simulink model "OCC_DQ_RCC_PO_BOOST_COMMON_GROUND_UPM"  (R2023a)
settings: Solver=ode1  StartTime=0.0  StopTime=5  FixedStep=1e-6  MaxStep=1e-6  RelTol=1e-3  EnableMultiTasking=on
undefined symbols (not defined in the file or in its folder): DiscIntNeverNeededParam
libraries: simulink x15, spsSeriesRLCBranchLib x14, spsVoltageMeasurementLib x8, slpidlib x7, spsDiodeLib x6, spsFirstOrderFilterLib x6, spsMosfetLib x5, powerlib_extras x5, spsCurrentMeasurementLib x4, spsAlphaBetaZerotodq0Lib x3, eePowerMeasurement x2, spsACVoltageSourceLib x1
(part 1 of 2)
Description:
  | Model of a simple control system for use iin training.
settings Model: Creator=Paul Baracos  LastModifiedBy=RAGHAVA
settings SolverCC: AutoInsertRateTranBlk=on
settings DataIOCC: LimitDataPoints=on  SaveFormat=StructureWithTime  SignalLoggingSaveFormat=ModelDataLogs  SaveOutput=off  SaveTime=off  ReturnWorkspaceOutputs=off  SignalLoggingName=sigsOut
settings OptimizationCC: BlockReduction=off  BooleanDataType=off  OptimizeBlockIOStorage=off  BufferReuse=off  ExpressionFolding=off  ExpressionDepthLimit=2147483647  LocalBlockOutputs=off  InitFltsAndDblsToZero=on  LifeSpan=inf
settings DebuggingCC: SaveWithParameterizedLinksMsg=none  UnderspecifiedInitializationDetection=Classic  MergeDetectMultiDrivingBlocksExec=none  SignalResolutionControl=TryResolveAllWithWarning  MultiTaskDSMMsg=warning  MultiTaskCondExecSysMsg=none  FcnCallInpInsideContextMsg=warning  UnconnectedInputMsg=warning  UnconnectedOutputMsg=warning  UnconnectedLineMsg=warning  StateNameClashWarn=warning  SFUnexpectedBacktrackingDiag=warning  SFNoUnconditionalDefaultTransitionDiag=warning  SFExecutionAtInitializationDiag=none  ArithmeticOperatorsInVariantConditions=warning
settings HardwareCC: ProdBitPerPointer=32  ProdBitPerSizeT=32  ProdBitPerPtrDiffT=32  ProdLargestAtomicFloat=None  ProdIntDivRoundTo=Undefined  ProdEndianess=Unspecified  ProdWordSize=32  ProdHWDeviceType=32-bit Generic  TargetBitPerPointer=64  TargetBitPerSizeT=64  TargetBitPerPtrDiffT=64  TargetLongLongMode=on  TargetIntDivRoundTo=Zero  TargetEndianess=LittleEndian  TargetWordSize=64  TargetHWDeviceType=MATLAB Host  ProdEqTarget=off
settings ModelReferenceCC: PropagateSignalLabelsOutOfModel=off
settings SFSimCC: SimUseLocalCustomCode=off  CustomCodeUndefinedFunction=UseInterfaceOnly
settings RTWCC: RTWUseLocalCustomCode=off
settings CodeAppCC: StateflowObjectComments=on
settings GRTTargetCC: TargetFcnLib=ansi_tfl_tmw.mat  TargetLangStandard=C89/C90 (ANSI)  CombineOutputUpdateFcns=off  GRTInterface=on
settings ConfigComp: CovMetricSettings=dw  CovSaveCumulativeToWorkspaceVar=on  CovSaveSingleToWorkspaceVar=on  CovExternalEMLEnable=off

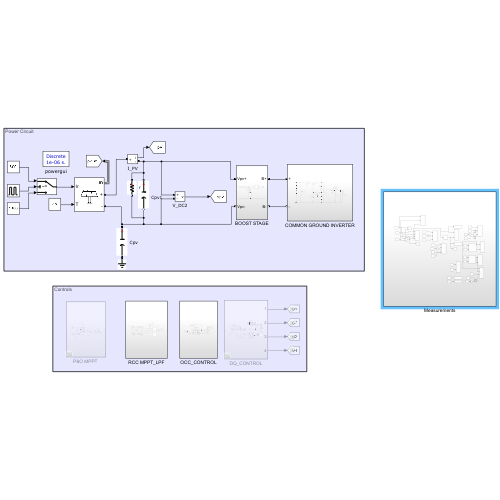
[thumbnail: Simulink's stored preview of the top-level diagram]
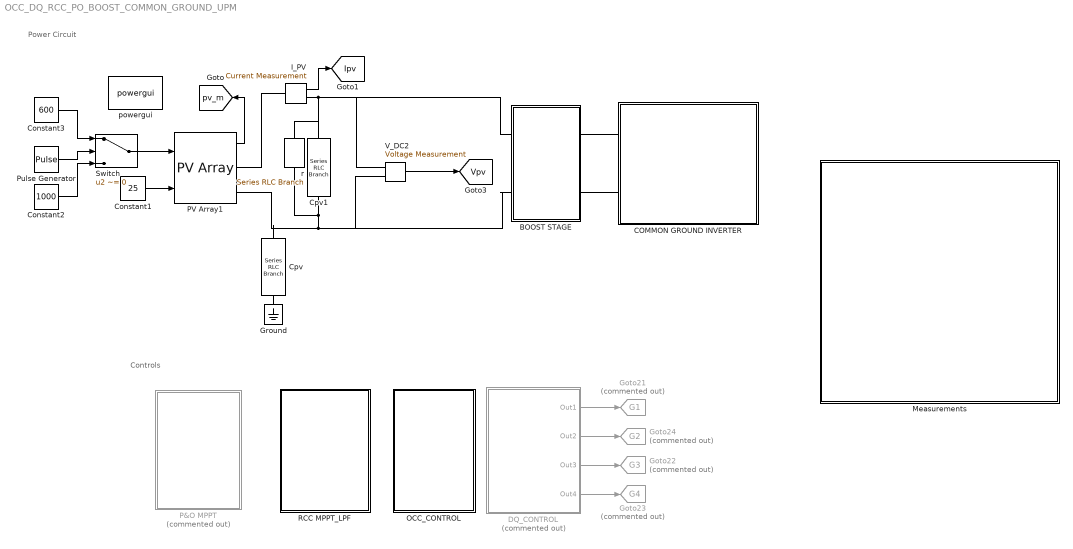
== system OCC_DQ_RCC_PO_BOOST_COMMON_GROUND_UPM ==
  note: Controls
  note: Power Circuit
  " Cpv1" : spsSeriesRLCBranchLib/Series RLC Branch  LConnTagsString=__new0  RConnTagsString=__new0  BranchType=C  Resistance=1  Inductance=15.5e-3  SetiL0=off  InitialCurrent=0  Capacitance=10e-6  Setx0=on  InitialVoltage=130  Measurements=Branch voltage and current
  BOOST STAGE : Subsystem
  COMMON GROUND INVERTER : Subsystem
  Constant1 : Constant  Value=25  SampleTime=0
  Constant2 : Constant  Value=1000
  Constant3 : Constant  Value=600
  Cpv : spsSeriesRLCBranchLib/Series RLC Branch  LConnTagsString=__new0  RConnTagsString=__new0  BranchType=C  Resistance=0.0001  Inductance=15.5e-3  SetiL0=off  InitialCurrent=0  Capacitance=100e-9  Setx0=off  InitialVoltage=0  Measurements=Branch voltage and current
  DQ_CONTROL : Subsystem  Commented=on
  Goto21 : Goto  Commented=on  GotoTag=G1  TagVisibility=global
  Goto22 : Goto  Commented=on  GotoTag=G3  TagVisibility=global
  Goto23 : Goto  Commented=on  GotoTag=G4  TagVisibility=global
  Goto24 : Goto  Commented=on  GotoTag=G2  TagVisibility=global
  Ground : spsGroundLib/Ground  LConnTagsString=a
  I_PV : spsCurrentMeasurementLib/Current Measurement  PhasorSimulation=off  OutputType=Complex  PSBequivalent=0
  Measurements : Subsystem
  OCC_CONTROL : Subsystem
  "P&O MPPT " : Subsystem  Commented=on
  PV Array1 : spsPVArrayLib/PV Array  Npar=1  Nser=5  PlotType=array @ 25 deg.C & specified irradiances  S_vec="[ 1000  600  100 ]"  Temp_C_vec="[ 45 25  ]"  ModuleName=Kyocera Solar KC200GT  PlotWhenSelected=off  Pm=200.143  Ncell=54  Voc=32.9  Isc=8.21  Vm=26.3  Im=7.61  beta_Voc_pc=-0.355  alpha_Isc_pc=0.06  beta_Voc=-0.11679  alpha_Isc=0.004926  IL=8.2288  I0=2.3234e-10  nI=0.97734  Rsh=150.6844  Rs=0.34484  RobustModel=off  RobustCellTemperature=313.3991  BAL=on  Tc=1e-6  Tfilter=5e-5
  Pulse Generator : DiscretePulseGenerator  PulseType=Time based  PulseWidth=50
  RCC MPPT_LPF : Subsystem
  Switch : Switch  Criteria=u2 ~= 0  SaturateOnIntegerOverflow=off  InputSameDT=off
  V_DC2 : spsVoltageMeasurementLib/Voltage Measurement  PhasorSimulation=off  OutputType=Complex  PSBequivalent=0
  powergui : sps_lib/powergui  Priority=1  SimulationMode=Discrete  SampleTime=1e-6  frequency=60  Iterations=50  frequencyindice=0  Pbase=100e6  ErrMax=1e-4  UnitsV=kV  UnitsW=MW  buscounter=0  FunctionMessages=off  echomessages=off  EnableUseOfTLC=off  CurrentSourceSwitches=off  DisableSnubberDevices=on  DisableRonSwitches=on  DisableVfSwitches=on  DisplayEquations=off  AutomaticDiscreteSolvers=off  SolverType=Tustin/Backward Euler (TBE)  Interpol=off  ExternalGateDelay=off  methode=off  Ts=0  x0status=blocks  SPID=on  SwTol=0  HookPort=off  NonlinearTolerance=1e-4  nMaxIteration=100  ContinueOnMaxIteration=off  RestoreLinks=warning  ResistiveCurrentMeasurement=off  Frange=[0:2:500]  Ylog=off  Xlog=on  ShowGrid=off  save=off  variable=ZData  structure=0  ZoomFFT=off  StartTime=0.0  cycles=1  DisplayStyle=1  fundamental=60  FreqAxis=off  MaxFrequency=1000  frequencyindicesteady=1  RmsSteady=1  display=off
  r : spsSeriesRLCBranchLib/Series RLC Branch  LConnTagsString=__new0  RConnTagsString=__new0  BranchType=R  Resistance=10000  Inductance=15.5e-3  SetiL0=off  InitialCurrent=0  Capacitance=2200e-6  Setx0=off  InitialVoltage=0  Measurements=Branch voltage and current
  tag scope: Ipv=global, Vpv=global, pv_m=global
  wires:
  Pulse Generator/1 -> Switch/2
  I_PV/1 -> [Ipv]
  Constant1/1 -> PV Array1/2
  V_DC2/1 -> [Vpv]
  PV Array1/1 -> [pv_m]
  DQ_CONTROL/3(Out3) -> Goto22/1
  DQ_CONTROL/2(Out2) -> Goto24/1
  DQ_CONTROL/4(Out4) -> Goto23/1
  DQ_CONTROL/1(Out1) -> Goto21/1
  Constant2/1 -> Switch/3
  Constant3/1 -> Switch/1
  Switch/1 -> PV Array1/1
  connections:
  PV Array1/RConn1 -- I_PV/LConn1
  I_PV/RConn1 -- r/LConn1 -- " Cpv1"/LConn1 -- V_DC2/LConn1 -- BOOST STAGE/LConn1
  " Cpv1"/RConn1 -- r/RConn1 -- Cpv/LConn1 -- PV Array1/RConn2 -- V_DC2/LConn2 -- BOOST STAGE/LConn2
  COMMON GROUND INVERTER/LConn1 -- BOOST STAGE/RConn1
  COMMON GROUND INVERTER/LConn2 -- BOOST STAGE/RConn2
  Ground/LConn1 -- Cpv/RConn1

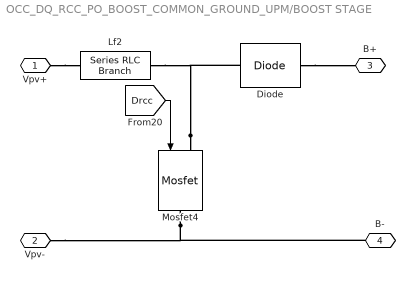
== system OCC_DQ_RCC_PO_BOOST_COMMON_GROUND_UPM/BOOST STAGE ==
  Diode : spsDiodeLib/Diode  Ron=0.001  Lon=0  Vf=0.8  IC=0  UseSnubber=0  Rs=500  Cs=250e-9  Measurements=off
  Lf2 : spsSeriesRLCBranchLib/Series RLC Branch  LConnTagsString=__new0  RConnTagsString=__new0  BranchType=RL  Resistance=0.0001  Inductance=5.87e-3  SetiL0=off  InitialCurrent=0  Capacitance=1e-6  Setx0=off  InitialVoltage=0  Measurements=Branch voltage and current
  Mosfet4 : spsMosfetLib/Mosfet  Ron=0.001  Lon=0  Rd=0.001  Vfd=0.8  IC=0  Rs=1e9  Cs=inf  Measurements=off
  Vpv+ : PMIOPort  Side=Left
  Vpv- : PMIOPort  Port=2  Side=Left
  B+ : PMIOPort  Port=3  Side=Right
  B- : PMIOPort  Port=4  Side=Right
  wires:
  [Drcc] -> Mosfet4/1
  connections:
  Diode/RConn1 -- B+/RConn1
  Vpv+/RConn1 -- Lf2/LConn1
  Mosfet4/RConn1 -- B-/RConn1 -- Vpv-/RConn1
  Mosfet4/LConn1 -- Diode/LConn1 -- Lf2/RConn1

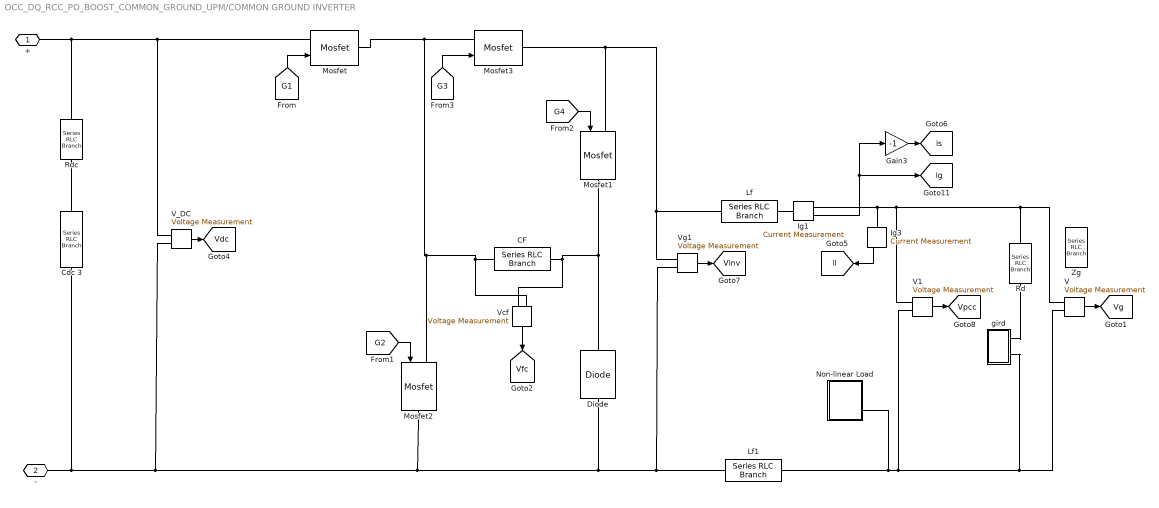
== system OCC_DQ_RCC_PO_BOOST_COMMON_GROUND_UPM/COMMON GROUND INVERTER ==
  CF : spsSeriesRLCBranchLib/Series RLC Branch  LConnTagsString=__new0  RConnTagsString=__new0  BranchType=C  Resistance=0.0001  Inductance=15.5e-3  SetiL0=off  InitialCurrent=0  Capacitance=1100e-6  Setx0=on  InitialVoltage=400  Measurements=Branch voltage and current
  Cdc 3 : spsSeriesRLCBranchLib/Series RLC Branch  LConnTagsString=__new0  RConnTagsString=__new0  BranchType=C  Resistance=0.0001  Inductance=15.5e-3  SetiL0=off  InitialCurrent=0  Capacitance=1000e-6  Setx0=on  InitialVoltage=400  Measurements=Branch voltage and current
  Diode : spsDiodeLib/Diode  Ron=0.001  Lon=0  Vf=0.8  IC=0  UseSnubber=0  Rs=500  Cs=250e-9  Measurements=off
  Gain3 : Gain  Gain=-1
  Ig1 : spsCurrentMeasurementLib/Current Measurement  PhasorSimulation=off  OutputType=Complex  PSBequivalent=0
  Ig3 : spsCurrentMeasurementLib/Current Measurement  PhasorSimulation=off  OutputType=Complex  PSBequivalent=0
  Lf : spsSeriesRLCBranchLib/Series RLC Branch  LConnTagsString=__new0  RConnTagsString=__new0  BranchType=RL  Resistance=0.01  Inductance=8e-3  SetiL0=off  InitialCurrent=0  Capacitance=1e-6  Setx0=off  InitialVoltage=0  Measurements=Branch voltage and current
  Lf1 : spsSeriesRLCBranchLib/Series RLC Branch  LConnTagsString=__new0  RConnTagsString=__new0  BranchType=RL  Resistance=0.01  Inductance=8e-3  SetiL0=off  InitialCurrent=0  Capacitance=1e-6  Setx0=off  InitialVoltage=0  Measurements=Branch voltage and current
  Mosfet{,1..3} (4 alike) : spsMosfetLib/Mosfet  Ron=0.001  Lon=0  Rd=0.001  Vfd=0.8  IC=0  Rs=1e9  Cs=inf  Measurements=off
  Non-linear Load : Subsystem
  Rd : spsSeriesRLCBranchLib/Series RLC Branch  LConnTagsString=__new0  RConnTagsString=__new0  BranchType=R  Resistance=0.08  Inductance=1.5e-3  SetiL0=off  InitialCurrent=0  Capacitance=2200e-6  Setx0=off  InitialVoltage=0  Measurements=Branch voltage and current
  "Rdc " : spsSeriesRLCBranchLib/Series RLC Branch  LConnTagsString=__new0  RConnTagsString=__new0  BranchType=R  Resistance=0.0001  Inductance=15.5e-3  SetiL0=off  InitialCurrent=0  Capacitance=2200e-6  Setx0=off  InitialVoltage=0  Measurements=Branch voltage and current
  V : spsVoltageMeasurementLib/Voltage Measurement  PhasorSimulation=off  OutputType=Complex  PSBequivalent=0
  V1 : spsVoltageMeasurementLib/Voltage Measurement  PhasorSimulation=off  OutputType=Complex  PSBequivalent=0
  V_DC : spsVoltageMeasurementLib/Voltage Measurement  PhasorSimulation=off  OutputType=Complex  PSBequivalent=0
  Vcf : spsVoltageMeasurementLib/Voltage Measurement  PhasorSimulation=off  OutputType=Complex  PSBequivalent=0
  Vg1 : spsVoltageMeasurementLib/Voltage Measurement  PhasorSimulation=off  OutputType=Complex  PSBequivalent=0
  Zg : spsSeriesRLCBranchLib/Series RLC Branch  LConnTagsString=__new0  RConnTagsString=__new0  BranchType=RL  Resistance=0.08  Inductance=1.5e-3  SetiL0=off  InitialCurrent=0  Capacitance=2200e-6  Setx0=off  InitialVoltage=0  Measurements=Branch voltage and current
  gird : Subsystem
  + : PMIOPort  Side=Left
  - : PMIOPort  Port=2  Side=Left
  tag scope: Vdc=global, Vfc=global, Vg=global, Vinv=global, Vpcc=global, ig=global, il=global, is=global
  wires:
  [G2] -> Mosfet2/1
  Ig1/1 -> [ig], Gain3/1
  [G1] -> Mosfet/1
  Vg1/1 -> [Vinv]
  V_DC/1 -> [Vdc]
  V/1 -> [Vg]
  [G3] -> Mosfet3/1
  [G4] -> Mosfet1/1
  Gain3/1 -> [is]
  Vcf/1 -> [Vfc]
  Ig3/1 -> [il]
  V1/1 -> [Vpcc]
  connections:
  Vg1/LConn1 -- Mosfet1/LConn1 -- Mosfet3/RConn1 -- Lf/LConn1
  Ig1/LConn1 -- Lf/RConn1
  Cdc 3/LConn1 -- "Rdc "/RConn1
  "Rdc "/LConn1 -- +/RConn1 -- V_DC/LConn1 -- Mosfet/LConn1
  Mosfet3/LConn1 -- Vcf/LConn1 -- CF/LConn1 -- Mosfet2/LConn1 -- Mosfet/RConn1
  CF/RConn1 -- Diode/LConn1 -- Mosfet1/RConn1 -- Vcf/LConn2
  gird/LConn2 -- Non-linear Load/LConn2 -- Lf1/RConn1 -- V1/LConn2 -- V/LConn2
  Lf1/LConn1 -- Vg1/LConn2 -- Mosfet2/RConn1 -- V_DC/LConn2 -- -/RConn1 -- Cdc 3/RConn1 -- Diode/RConn1
  V/LConn1 -- V1/LConn1 -- Ig3/LConn1 -- Ig1/RConn1 -- Rd/LConn1
  Rd/RConn1 -- gird/LConn1

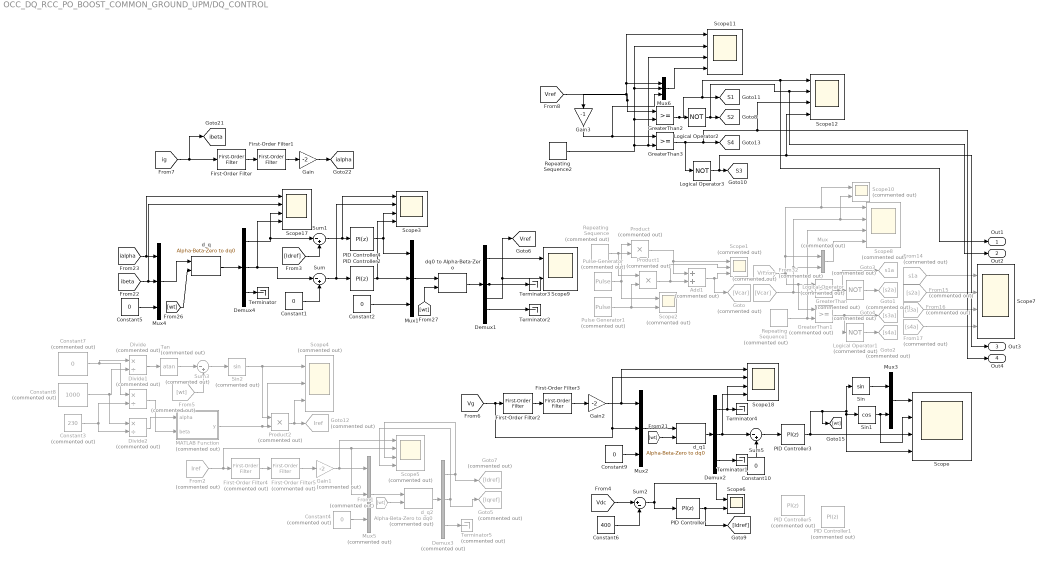
== system OCC_DQ_RCC_PO_BOOST_COMMON_GROUND_UPM/DQ_CONTROL ==
  Add1 : Sum  Commented=on
  Constant{1..2,5,9..10} (5 alike) : Constant  Value=0
  Constant3 : Constant  Commented=on  Value=230
  Constant4 : Constant  Commented=on  Value=0
  Constant6 : Constant  Value=400
  Constant7 : Constant  Commented=on  Value=0
  Constant8 : Constant  Commented=on  Value=1000
  Demux1 : Demux  Outputs=3
  Demux2 : Demux  Outputs=3
  Demux3 : Demux  Commented=on  Outputs=3
  Demux4 : Demux  Outputs=3
  Divide : Product  Commented=on  Inputs=*/  RndMeth=Zero  SaturateOnIntegerOverflow=on
  Divide1 : Product  Commented=on  Inputs=*/  RndMeth=Zero  SaturateOnIntegerOverflow=on
  Divide2 : Product  Commented=on  Inputs=*/  RndMeth=Zero  SaturateOnIntegerOverflow=on
  First-Order Filter : spsFirstOrderFilterLib/First-Order Filter  FilterType=Lowpass  Tc=1/(2*pi*50)  Ts=1e-6  Initialize=off  Vac_Init=[0, 0, 60]  Vdc_Init=0  PlotResponse=off  FreqRange="[0,  200,  1]"
  First-Order Filter1 : spsFirstOrderFilterLib/First-Order Filter  FilterType=Lowpass  Tc=1/(2*pi*50)  Ts=1e-6  Initialize=off  Vac_Init=[0, 0, 60]  Vdc_Init=0  PlotResponse=off  FreqRange="[0,  200,  1]"
  First-Order Filter2 : spsFirstOrderFilterLib/First-Order Filter  FilterType=Lowpass  Tc=1/(2*pi*50)  Ts=1e-6  Initialize=off  Vac_Init=[0, 0, 50]  Vdc_Init=0  PlotResponse=off  FreqRange="[0,  200,  1]"
  First-Order Filter3 : spsFirstOrderFilterLib/First-Order Filter  FilterType=Lowpass  Tc=1/(2*pi*50)  Ts=1e-6  Initialize=off  Vac_Init=[0, 0, 50]  Vdc_Init=0  PlotResponse=off  FreqRange="[0,  200,  1]"
  First-Order Filter4 : spsFirstOrderFilterLib/First-Order Filter  Commented=on  FilterType=Lowpass  Tc=1/(2*pi*50)  Ts=1e-6  Initialize=off  Vac_Init=[0, 0, 50]  Vdc_Init=0  PlotResponse=off  FreqRange="[0,  200,  1]"
  First-Order Filter5 : spsFirstOrderFilterLib/First-Order Filter  Commented=on  FilterType=Lowpass  Tc=1/(2*pi*50)  Ts=1e-6  Initialize=off  Vac_Init=[0, 0, 50]  Vdc_Init=0  PlotResponse=off  FreqRange="[0,  200,  1]"
  From : From  Commented=on  GotoTag=Vcar
  From1 : From  Commented=on  GotoTag=wt
  From14 : From  Commented=on  GotoTag=s1a  TagVisibility=global
  From15 : From  Commented=on  GotoTag=s2a
  From16 : From  Commented=on  GotoTag=s3a
  From17 : From  Commented=on  GotoTag=s4a
  From2 : From  Commented=on  GotoTag=Iref  TagVisibility=global
  From32 : From  Commented=on  GotoTag=Vref  TagVisibility=global
  From5 : From  Commented=on  GotoTag=wt
  Gain : Gain  Gain=-2
  Gain1 : Gain  Commented=on  Gain=-2
  Gain2 : Gain  Gain=-2
  Gain3 : Gain  Gain=-1
  Goto : Goto  Commented=on  GotoTag=Vcar
  Goto1 : Goto  Commented=on  GotoTag=s2a
  Goto12 : Goto  Commented=on  GotoTag=Iref  TagVisibility=global
  Goto2 : Goto  Commented=on  GotoTag=s4a
  Goto3 : Goto  Commented=on  GotoTag=s1a  TagVisibility=global
  Goto4 : Goto  Commented=on  GotoTag=s3a
  Goto5 : Goto  Commented=on  GotoTag=Iqref
  Goto7 : Goto  Commented=on  GotoTag=Idref
  GreaterThan : RelationalOperator  Commented=on  OutDataTypeStr=boolean  RndMeth=Simplest  InputSameDT=off
  GreaterThan1 : RelationalOperator  Commented=on  OutDataTypeStr=boolean  RndMeth=Simplest  InputSameDT=off
  GreaterThan2 : RelationalOperator  OutDataTypeStr=boolean  RndMeth=Simplest  InputSameDT=off
  GreaterThan3 : RelationalOperator  OutDataTypeStr=boolean  RndMeth=Simplest  InputSameDT=off
  Logical Operator : Logic  Commented=on  Operator=NOT  AllPortsSameDT=off  OutDataTypeStr=boolean
  Logical Operator1 : Logic  Commented=on  Operator=NOT  AllPortsSameDT=off  OutDataTypeStr=boolean
  Logical Operator2 : Logic  Operator=NOT  AllPortsSameDT=off  OutDataTypeStr=boolean
  Logical Operator3 : Logic  Operator=NOT  AllPortsSameDT=off  OutDataTypeStr=boolean
  MATLAB Function : MATLAB Function  Commented=on  TreatAsAtomicUnit=on
  Mux : Mux  Commented=on  Inputs=2
  Mux{1..2,4,6} (4 alike) : Mux  Inputs=3
  Mux3 : Mux  Inputs=2
  Mux5 : Mux  Commented=on  Inputs=3
  PID Controller : slpidlib/PID Controller  Controller=PI  Form=Parallel  TimeDomain=Discrete-time  UseExternalTs=off  SampleTime=-1  IntegratorMethod=Forward Euler  FilterMethod=Forward Euler  ControllerParametersSource=internal  P=1/(65.15*0.45)*5  I=0.4  UseKiTs=off  D=0  N=100  UseFilter=on  TunerSelectOption=Transfer Function Based (PID Tuner App)  InitialConditionSource=internal  InitialConditionForIntegrator=0  InitialConditionForFilter=0  DifferentiatorICPrevScaledInput=0  ExternalReset=none  TrackingMode=off  Kt=1  LimitOutput=off  SatLimitsSource=internal  UpperSaturationLimit=inf  LowerSaturationLimit=-inf  LinearizeAsGain=on  AntiWindupMode=none  Kb=1  LimitIntegrator=off  UpperIntegratorSaturationLimit=inf  LowerIntegratorSaturationLimit=-inf  POutMin=[]  POutMax=[]  IOutMin=[]  IOutMax=[]  DOutMin=[]  DOutMax=[]  NOutMin=[]  NOutMax=[]  SumOutMin=[]  SumOutMax=[]  SaturationOutMin=[]  SaturationOutMax=[]  PParamMin=[]  PParamMax=[]  IParamMin=[]  IParamMax=[]  DParamMin=[]  DParamMax=[]  NParamMin=[]  NParamMax=[]  KbParamMin=[]  KbParamMax=[]  KtParamMin=[]  KtParamMax=[]  KbOutMin=[]  KbOutMax=[]  KtOutMin=[]  KtOutMax=[]  IntegratorOutMin=[]  IntegratorOutMax=[]  FilterOutMin=[]  FilterOutMax=[]  SumI1OutMin=[]  SumI1OutMax=[]  SumI2OutMin=[]  SumI2OutMax=[]  SumI3OutMin=[]  SumI3OutMax=[]  SumI4OutMin=[]  SumI4OutMax=[]  SumDOutMin=[]  SumDOutMax=[]  DifferentiatorOutMin=[]  DifferentiatorOutMax=[]  FilterDiffOutCoefMin=[]  FilterDiffOutCoefMax=[]  ReciprocalOutMin=[]  ReciprocalOutMax=[]  SumDenOutMin=[]  SumDenOutMax=[]  SumNumOutMin=[]  SumNumOutMax=[]  DivideOutMin=[]  DivideOutMax=[]  UdiffTsProdOutMin=[]  UdiffTsProdOutMax=[]  NTsProdOutMin=[]  NTsProdOutMax=[]  UintegralTsProdOutMin=[]  UintegralTsProdOutMax=[]  UngainTsProdOutMin=[]  UngainTsProdOutMax=[]  ClampingZeroOutDataTypeStr=Inherit: Inherit via back propagation  ClampingZeroOutMin=[]  ClampingZeroOutMax=[]  FilterDenConstantOutDataTypeStr=Inherit: Inherit via back propagation  FilterDenConstantOutMin=[]  FilterDenConstantOutMax=[]  PCopyOutDataTypeStr=Inherit: Inherit via back propagation  PCopyOutMin=[]  PCopyOutMax=[]  NCopyOutDataTypeStr=Inherit: Inherit via back propagation  NCopyOutMin=[]  NCopyOutMax=[]  IntegratorContinuousStateAttributes=''  IntegratorStateMustResolveToSignalObject=off  IntegratorRTWStateStorageClass=Auto  FilterContinuousStateAttributes=''  FilterStateMustResolveToSignalObject=off  FilterRTWStateStorageClass=Auto  ParallelPVariant=InternalParameters  IdealPVariant=Disabled  IVariant=InternalParameters  DVariant=Disabled  IntegratorVariant=Discrete  SatVariant=Disabled  AWVariant=Passthrough  PCopyVariant=Disabled  TRVariant=Disabled  FdbkBlocksVariant=Forward  IdealPFdbkVariant=Disabled  SatFdbkVariant=Disabled  DerivativeFilterVariant=Disabled  NVariant=Disabled  NCopyVariant=Disabled_SignalSpec  FilterICVariant=Disabled  IntegratorICVariant=InternalICs  ExternalResetVariant=Disabled  TRSumVariant=Passthrough  SumFdbkVariant=Disabled  SumVariant=Sum_PI  TsampFilterVariant=InternalTs  TsampNgainVariant=Passthrough  TsampIntegralVariant=Disabled_SignalSpec  ExternalSaturationOutDataTypeStr=Inherit: Same as second input
  PID Controller1 : slpidlib/PID Controller  Commented=on  Controller=PI  Form=Parallel  TimeDomain=Discrete-time  UseExternalTs=off  SampleTime=-1  IntegratorMethod=Forward Euler  FilterMethod=Forward Euler  ControllerParametersSource=internal  P=0.02*0.45*4*3  I=1  UseKiTs=off  D=0  N=100  UseFilter=on  TunerSelectOption=Transfer Function Based (PID Tuner App)  InitialConditionSource=internal  InitialConditionForIntegrator=0  InitialConditionForFilter=0  DifferentiatorICPrevScaledInput=0  ExternalReset=none  TrackingMode=off  Kt=1  LimitOutput=off  SatLimitsSource=internal  UpperSaturationLimit=inf  LowerSaturationLimit=-inf  LinearizeAsGain=on  AntiWindupMode=none  Kb=1  LimitIntegrator=off  UpperIntegratorSaturationLimit=inf  LowerIntegratorSaturationLimit=-inf  POutMin=[]  POutMax=[]  IOutMin=[]  IOutMax=[]  DOutMin=[]  DOutMax=[]  NOutMin=[]  NOutMax=[]  SumOutMin=[]  SumOutMax=[]  SaturationOutMin=[]  SaturationOutMax=[]  PParamMin=[]  PParamMax=[]  IParamMin=[]  IParamMax=[]  DParamMin=[]  DParamMax=[]  NParamMin=[]  NParamMax=[]  KbParamMin=[]  KbParamMax=[]  KtParamMin=[]  KtParamMax=[]  KbOutMin=[]  KbOutMax=[]  KtOutMin=[]  KtOutMax=[]  IntegratorOutMin=[]  IntegratorOutMax=[]  FilterOutMin=[]  FilterOutMax=[]  SumI1OutMin=[]  SumI1OutMax=[]  SumI2OutMin=[]  SumI2OutMax=[]  SumI3OutMin=[]  SumI3OutMax=[]  SumI4OutMin=[]  SumI4OutMax=[]  SumDOutMin=[]  SumDOutMax=[]  DifferentiatorOutMin=[]  DifferentiatorOutMax=[]  FilterDiffOutCoefMin=[]  FilterDiffOutCoefMax=[]  ReciprocalOutMin=[]  ReciprocalOutMax=[]  SumDenOutMin=[]  SumDenOutMax=[]  SumNumOutMin=[]  SumNumOutMax=[]  DivideOutMin=[]  DivideOutMax=[]  UdiffTsProdOutMin=[]  UdiffTsProdOutMax=[]  NTsProdOutMin=[]  NTsProdOutMax=[]  UintegralTsProdOutMin=[]  UintegralTsProdOutMax=[]  UngainTsProdOutMin=[]  UngainTsProdOutMax=[]  ClampingZeroOutDataTypeStr=Inherit: Inherit via back propagation  ClampingZeroOutMin=[]  ClampingZeroOutMax=[]  FilterDenConstantOutDataTypeStr=Inherit: Inherit via back propagation  FilterDenConstantOutMin=[]  FilterDenConstantOutMax=[]  PCopyOutDataTypeStr=Inherit: Inherit via back propagation  PCopyOutMin=[]  PCopyOutMax=[]  NCopyOutDataTypeStr=Inherit: Inherit via back propagation  NCopyOutMin=[]  NCopyOutMax=[]  IntegratorContinuousStateAttributes=''  IntegratorStateMustResolveToSignalObject=off  IntegratorRTWStateStorageClass=Auto  FilterContinuousStateAttributes=''  FilterStateMustResolveToSignalObject=off  FilterRTWStateStorageClass=Auto  ParallelPVariant=InternalParameters  IdealPVariant=Disabled  IVariant=InternalParameters  DVariant=Disabled  IntegratorVariant=Discrete  SatVariant=Disabled  AWVariant=Passthrough  PCopyVariant=Disabled  TRVariant=Disabled  FdbkBlocksVariant=Forward  IdealPFdbkVariant=Disabled  SatFdbkVariant=Disabled  DerivativeFilterVariant=Disabled  NVariant=Disabled  NCopyVariant=Disabled_SignalSpec  FilterICVariant=Disabled  IntegratorICVariant=InternalICs  ExternalResetVariant=Disabled  TRSumVariant=Passthrough  SumFdbkVariant=Disabled  SumVariant=Sum_PI  TsampFilterVariant=InternalTs  TsampNgainVariant=Passthrough  TsampIntegralVariant=Disabled_SignalSpec  ExternalSaturationOutDataTypeStr=Inherit: Same as second input
  PID Controller2 : slpidlib/PID Controller  Controller=PI  Form=Parallel  TimeDomain=Discrete-time  UseExternalTs=off  SampleTime=-1  IntegratorMethod=Forward Euler  FilterMethod=Forward Euler  ControllerParametersSource=internal  P=0.05*0.45*4  I=0.05*0.45/0.02*4  UseKiTs=off  D=0  N=100  UseFilter=on  TunerSelectOption=Transfer Function Based (PID Tuner App)  InitialConditionSource=internal  InitialConditionForIntegrator=0  InitialConditionForFilter=0  DifferentiatorICPrevScaledInput=0  ExternalReset=none  TrackingMode=off  Kt=1  LimitOutput=off  SatLimitsSource=internal  UpperSaturationLimit=inf  LowerSaturationLimit=-inf  LinearizeAsGain=on  AntiWindupMode=none  Kb=1  LimitIntegrator=off  UpperIntegratorSaturationLimit=inf  LowerIntegratorSaturationLimit=-inf  POutMin=[]  POutMax=[]  IOutMin=[]  IOutMax=[]  DOutMin=[]  DOutMax=[]  NOutMin=[]  NOutMax=[]  SumOutMin=[]  SumOutMax=[]  SaturationOutMin=[]  SaturationOutMax=[]  PParamMin=[]  PParamMax=[]  IParamMin=[]  IParamMax=[]  DParamMin=[]  DParamMax=[]  NParamMin=[]  NParamMax=[]  KbParamMin=[]  KbParamMax=[]  KtParamMin=[]  KtParamMax=[]  KbOutMin=[]  KbOutMax=[]  KtOutMin=[]  KtOutMax=[]  IntegratorOutMin=[]  IntegratorOutMax=[]  FilterOutMin=[]  FilterOutMax=[]  SumI1OutMin=[]  SumI1OutMax=[]  SumI2OutMin=[]  SumI2OutMax=[]  SumI3OutMin=[]  SumI3OutMax=[]  SumI4OutMin=[]  SumI4OutMax=[]  SumDOutMin=[]  SumDOutMax=[]  DifferentiatorOutMin=[]  DifferentiatorOutMax=[]  FilterDiffOutCoefMin=[]  FilterDiffOutCoefMax=[]  ReciprocalOutMin=[]  ReciprocalOutMax=[]  SumDenOutMin=[]  SumDenOutMax=[]  SumNumOutMin=[]  SumNumOutMax=[]  DivideOutMin=[]  DivideOutMax=[]  UdiffTsProdOutMin=[]  UdiffTsProdOutMax=[]  NTsProdOutMin=[]  NTsProdOutMax=[]  UintegralTsProdOutMin=[]  UintegralTsProdOutMax=[]  UngainTsProdOutMin=[]  UngainTsProdOutMax=[]  ClampingZeroOutDataTypeStr=Inherit: Inherit via back propagation  ClampingZeroOutMin=[]  ClampingZeroOutMax=[]  FilterDenConstantOutDataTypeStr=Inherit: Inherit via back propagation  FilterDenConstantOutMin=[]  FilterDenConstantOutMax=[]  PCopyOutDataTypeStr=Inherit: Inherit via back propagation  PCopyOutMin=[]  PCopyOutMax=[]  NCopyOutDataTypeStr=Inherit: Inherit via back propagation  NCopyOutMin=[]  NCopyOutMax=[]  IntegratorContinuousStateAttributes=''  IntegratorStateMustResolveToSignalObject=off  IntegratorRTWStateStorageClass=Auto  FilterContinuousStateAttributes=''  FilterStateMustResolveToSignalObject=off  FilterRTWStateStorageClass=Auto  ParallelPVariant=InternalParameters  IdealPVariant=Disabled  IVariant=InternalParameters  DVariant=Disabled  IntegratorVariant=Discrete  SatVariant=Disabled  AWVariant=Passthrough  PCopyVariant=Disabled  TRVariant=Disabled  FdbkBlocksVariant=Forward  IdealPFdbkVariant=Disabled  SatFdbkVariant=Disabled  DerivativeFilterVariant=Disabled  NVariant=Disabled  NCopyVariant=Disabled_SignalSpec  FilterICVariant=Disabled  IntegratorICVariant=InternalICs  ExternalResetVariant=Disabled  TRSumVariant=Passthrough  SumFdbkVariant=Disabled  SumVariant=Sum_PI  TsampFilterVariant=InternalTs  TsampNgainVariant=Passthrough  TsampIntegralVariant=Disabled_SignalSpec  ExternalSaturationOutDataTypeStr=Inherit: Same as second input
  PID Controller3 : slpidlib/PID Controller  Controller=PI  Form=Parallel  TimeDomain=Discrete-time  UseExternalTs=off  SampleTime=-1  IntegratorMethod=Forward Euler  FilterMethod=Forward Euler  ControllerParametersSource=internal  P=-10  I=-50000  UseKiTs=off  D=1  N=100  UseFilter=on  TunerSelectOption=Frequency Response Based  ZeroCross=off  InitialConditionSource=internal  InitialConditionForIntegrator=0  InitialConditionForFilter=0  DifferentiatorICPrevScaledInput=0  ExternalReset=none  TrackingMode=off  Kt=1  LimitOutput=off  SatLimitsSource=internal  UpperSaturationLimit=inf  LowerSaturationLimit=-inf  LinearizeAsGain=on  AntiWindupMode=none  Kb=1  LimitIntegrator=off  UpperIntegratorSaturationLimit=inf  LowerIntegratorSaturationLimit=-inf  POutMin=[]  POutMax=[]  IOutMin=[]  IOutMax=[]  DOutMin=[]  DOutMax=[]  NOutMin=[]  NOutMax=[]  SumOutMin=[]  SumOutMax=[]  SaturationOutMin=[]  SaturationOutMax=[]  PParamMin=[]  PParamMax=[]  IParamMin=[]  IParamMax=[]  DParamMin=[]  DParamMax=[]  NParamMin=[]  NParamMax=[]  KbParamMin=[]  KbParamMax=[]  KtParamMin=[]  KtParamMax=[]  KbOutMin=[]  KbOutMax=[]  KtOutMin=[]  KtOutMax=[]  IntegratorOutMin=[]  IntegratorOutMax=[]  FilterOutMin=[]  FilterOutMax=[]  SumI1OutMin=[]  SumI1OutMax=[]  SumI2OutMin=[]  SumI2OutMax=[]  SumI3OutMin=[]  SumI3OutMax=[]  SumI4OutMin=[]  SumI4OutMax=[]  SumDOutMin=[]  SumDOutMax=[]  DifferentiatorOutMin=[]  DifferentiatorOutMax=[]  FilterDiffOutCoefMin=[]  FilterDiffOutCoefMax=[]  ReciprocalOutMin=[]  ReciprocalOutMax=[]  SumDenOutMin=[]  SumDenOutMax=[]  SumNumOutMin=[]  SumNumOutMax=[]  DivideOutMin=[]  DivideOutMax=[]  UdiffTsProdOutMin=[]  UdiffTsProdOutMax=[]  NTsProdOutMin=[]  NTsProdOutMax=[]  UintegralTsProdOutMin=[]  UintegralTsProdOutMax=[]  UngainTsProdOutMin=[]  UngainTsProdOutMax=[]  ClampingZeroOutDataTypeStr=Inherit: Inherit via back propagation  ClampingZeroOutMin=[]  ClampingZeroOutMax=[]  FilterDenConstantOutDataTypeStr=Inherit: Inherit via back propagation  FilterDenConstantOutMin=[]  FilterDenConstantOutMax=[]  PCopyOutDataTypeStr=Inherit: Inherit via back propagation  PCopyOutMin=[]  PCopyOutMax=[]  NCopyOutDataTypeStr=Inherit: Inherit via back propagation  NCopyOutMin=[]  NCopyOutMax=[]  IntegratorContinuousStateAttributes=''  IntegratorStateMustResolveToSignalObject=off  IntegratorRTWStateStorageClass=Auto  FilterContinuousStateAttributes=''  FilterStateMustResolveToSignalObject=off  FilterRTWStateStorageClass=Auto  ParallelPVariant=InternalParameters  IdealPVariant=Disabled  IVariant=InternalParameters  DVariant=Disabled  IntegratorVariant=Discrete  SatVariant=Disabled  AWVariant=Passthrough  PCopyVariant=Disabled  TRVariant=Disabled  FdbkBlocksVariant=Forward  IdealPFdbkVariant=Disabled  SatFdbkVariant=Disabled  DerivativeFilterVariant=Disabled  NVariant=Disabled  NCopyVariant=Disabled_SignalSpec  FilterICVariant=Disabled  IntegratorICVariant=InternalICs  ExternalResetVariant=Disabled  TRSumVariant=Passthrough  SumFdbkVariant=Disabled  SumVariant=Sum_PI  TsampFilterVariant=InternalTs  TsampNgainVariant=Passthrough  TsampIntegralVariant=Disabled_SignalSpec  ExternalSaturationOutDataTypeStr=Inherit: Same as second input
  PID Controller4 : slpidlib/PID Controller  Controller=PI  Form=Parallel  TimeDomain=Discrete-time  UseExternalTs=off  SampleTime=-1  IntegratorMethod=Forward Euler  FilterMethod=Forward Euler  ControllerParametersSource=internal  P=0.05*0.45*4  I=0.05*0.45/0.02*4  UseKiTs=off  D=0  N=100  UseFilter=on  TunerSelectOption=Transfer Function Based (PID Tuner App)  InitialConditionSource=internal  InitialConditionForIntegrator=0  InitialConditionForFilter=0  DifferentiatorICPrevScaledInput=0  ExternalReset=none  TrackingMode=off  Kt=1  LimitOutput=off  SatLimitsSource=internal  UpperSaturationLimit=inf  LowerSaturationLimit=-inf  LinearizeAsGain=on  AntiWindupMode=none  Kb=1  LimitIntegrator=off  UpperIntegratorSaturationLimit=inf  LowerIntegratorSaturationLimit=-inf  POutMin=[]  POutMax=[]  IOutMin=[]  IOutMax=[]  DOutMin=[]  DOutMax=[]  NOutMin=[]  NOutMax=[]  SumOutMin=[]  SumOutMax=[]  SaturationOutMin=[]  SaturationOutMax=[]  PParamMin=[]  PParamMax=[]  IParamMin=[]  IParamMax=[]  DParamMin=[]  DParamMax=[]  NParamMin=[]  NParamMax=[]  KbParamMin=[]  KbParamMax=[]  KtParamMin=[]  KtParamMax=[]  KbOutMin=[]  KbOutMax=[]  KtOutMin=[]  KtOutMax=[]  IntegratorOutMin=[]  IntegratorOutMax=[]  FilterOutMin=[]  FilterOutMax=[]  SumI1OutMin=[]  SumI1OutMax=[]  SumI2OutMin=[]  SumI2OutMax=[]  SumI3OutMin=[]  SumI3OutMax=[]  SumI4OutMin=[]  SumI4OutMax=[]  SumDOutMin=[]  SumDOutMax=[]  DifferentiatorOutMin=[]  DifferentiatorOutMax=[]  FilterDiffOutCoefMin=[]  FilterDiffOutCoefMax=[]  ReciprocalOutMin=[]  ReciprocalOutMax=[]  SumDenOutMin=[]  SumDenOutMax=[]  SumNumOutMin=[]  SumNumOutMax=[]  DivideOutMin=[]  DivideOutMax=[]  UdiffTsProdOutMin=[]  UdiffTsProdOutMax=[]  NTsProdOutMin=[]  NTsProdOutMax=[]  UintegralTsProdOutMin=[]  UintegralTsProdOutMax=[]  UngainTsProdOutMin=[]  UngainTsProdOutMax=[]  ClampingZeroOutDataTypeStr=Inherit: Inherit via back propagation  ClampingZeroOutMin=[]  ClampingZeroOutMax=[]  FilterDenConstantOutDataTypeStr=Inherit: Inherit via back propagation  FilterDenConstantOutMin=[]  FilterDenConstantOutMax=[]  PCopyOutDataTypeStr=Inherit: Inherit via back propagation  PCopyOutMin=[]  PCopyOutMax=[]  NCopyOutDataTypeStr=Inherit: Inherit via back propagation  NCopyOutMin=[]  NCopyOutMax=[]  IntegratorContinuousStateAttributes=''  IntegratorStateMustResolveToSignalObject=off  IntegratorRTWStateStorageClass=Auto  FilterContinuousStateAttributes=''  FilterStateMustResolveToSignalObject=off  FilterRTWStateStorageClass=Auto  ParallelPVariant=InternalParameters  IdealPVariant=Disabled  IVariant=InternalParameters  DVariant=Disabled  IntegratorVariant=Discrete  SatVariant=Disabled  AWVariant=Passthrough  PCopyVariant=Disabled  TRVariant=Disabled  FdbkBlocksVariant=Forward  IdealPFdbkVariant=Disabled  SatFdbkVariant=Disabled  DerivativeFilterVariant=Disabled  NVariant=Disabled  NCopyVariant=Disabled_SignalSpec  FilterICVariant=Disabled  IntegratorICVariant=InternalICs  ExternalResetVariant=Disabled  TRSumVariant=Passthrough  SumFdbkVariant=Disabled  SumVariant=Sum_PI  TsampFilterVariant=InternalTs  TsampNgainVariant=Passthrough  TsampIntegralVariant=Disabled_SignalSpec  ExternalSaturationOutDataTypeStr=Inherit: Same as second input
  PID Controller5 : slpidlib/PID Controller  Commented=on  Controller=PI  Form=Parallel  TimeDomain=Discrete-time  UseExternalTs=off  SampleTime=-1  IntegratorMethod=Forward Euler  FilterMethod=Forward Euler  ControllerParametersSource=internal  P=1/140*7*0.01*0.45/2  I=1/140*7*0.1*0.45/0.025  UseKiTs=off  D=0  N=100  UseFilter=on  TunerSelectOption=Transfer Function Based (PID Tuner App)  InitialConditionSource=internal  InitialConditionForIntegrator=0  InitialConditionForFilter=0  DifferentiatorICPrevScaledInput=0  ExternalReset=none  TrackingMode=off  Kt=1  LimitOutput=off  SatLimitsSource=internal  UpperSaturationLimit=inf  LowerSaturationLimit=-inf  LinearizeAsGain=on  AntiWindupMode=none  Kb=1  LimitIntegrator=off  UpperIntegratorSaturationLimit=inf  LowerIntegratorSaturationLimit=-inf  POutMin=[]  POutMax=[]  IOutMin=[]  IOutMax=[]  DOutMin=[]  DOutMax=[]  NOutMin=[]  NOutMax=[]  SumOutMin=[]  SumOutMax=[]  SaturationOutMin=[]  SaturationOutMax=[]  PParamMin=[]  PParamMax=[]  IParamMin=[]  IParamMax=[]  DParamMin=[]  DParamMax=[]  NParamMin=[]  NParamMax=[]  KbParamMin=[]  KbParamMax=[]  KtParamMin=[]  KtParamMax=[]  KbOutMin=[]  KbOutMax=[]  KtOutMin=[]  KtOutMax=[]  IntegratorOutMin=[]  IntegratorOutMax=[]  FilterOutMin=[]  FilterOutMax=[]  SumI1OutMin=[]  SumI1OutMax=[]  SumI2OutMin=[]  SumI2OutMax=[]  SumI3OutMin=[]  SumI3OutMax=[]  SumI4OutMin=[]  SumI4OutMax=[]  SumDOutMin=[]  SumDOutMax=[]  DifferentiatorOutMin=[]  DifferentiatorOutMax=[]  FilterDiffOutCoefMin=[]  FilterDiffOutCoefMax=[]  ReciprocalOutMin=[]  ReciprocalOutMax=[]  SumDenOutMin=[]  SumDenOutMax=[]  SumNumOutMin=[]  SumNumOutMax=[]  DivideOutMin=[]  DivideOutMax=[]  UdiffTsProdOutMin=[]  UdiffTsProdOutMax=[]  NTsProdOutMin=[]  NTsProdOutMax=[]  UintegralTsProdOutMin=[]  UintegralTsProdOutMax=[]  UngainTsProdOutMin=[]  UngainTsProdOutMax=[]  ClampingZeroOutDataTypeStr=Inherit: Inherit via back propagation  ClampingZeroOutMin=[]  ClampingZeroOutMax=[]  FilterDenConstantOutDataTypeStr=Inherit: Inherit via back propagation  FilterDenConstantOutMin=[]  FilterDenConstantOutMax=[]  PCopyOutDataTypeStr=Inherit: Inherit via back propagation  PCopyOutMin=[]  PCopyOutMax=[]  NCopyOutDataTypeStr=Inherit: Inherit via back propagation  NCopyOutMin=[]  NCopyOutMax=[]  IntegratorContinuousStateAttributes=''  IntegratorStateMustResolveToSignalObject=off  IntegratorRTWStateStorageClass=Auto  FilterContinuousStateAttributes=''  FilterStateMustResolveToSignalObject=off  FilterRTWStateStorageClass=Auto  ParallelPVariant=InternalParameters  IdealPVariant=Disabled  IVariant=InternalParameters  DVariant=Disabled  IntegratorVariant=Discrete  SatVariant=Disabled  AWVariant=Passthrough  PCopyVariant=Disabled  TRVariant=Disabled  FdbkBlocksVariant=Forward  IdealPFdbkVariant=Disabled  SatFdbkVariant=Disabled  DerivativeFilterVariant=Disabled  NVariant=Disabled  NCopyVariant=Disabled_SignalSpec  FilterICVariant=Disabled  IntegratorICVariant=InternalICs  ExternalResetVariant=Disabled  TRSumVariant=Passthrough  SumFdbkVariant=Disabled  SumVariant=Sum_PI  TsampFilterVariant=InternalTs  TsampNgainVariant=Passthrough  TsampIntegralVariant=Disabled_SignalSpec  ExternalSaturationOutDataTypeStr=Inherit: Same as second input
  Product : Product  Commented=on
  Product1 : Product  Commented=on
  Product2 : Product  Commented=on
  Pulse Generator : DiscretePulseGenerator  Commented=on  PulseType=Time based  Period=0.02  PulseWidth=50
  Pulse Generator1 : DiscretePulseGenerator  Commented=on  PulseType=Time based  Amplitude=-1  Period=0.02  PulseWidth=50  PhaseDelay=0.01
  Repeating Sequence : simulink/Sources/Repeating Sequence  Commented=on  rep_seq_t=[0 0.5 1]*1/10000  rep_seq_y=[0 1 0]
  Repeating Sequence1 : simulink/Sources/Repeating Sequence  Commented=on  rep_seq_t=[0 0.02]  rep_seq_y=[-1 1]
  Repeating Sequence2 : simulink/Sources/Repeating Sequence  rep_seq_t=[0 0.5 1]*1/10000  rep_seq_y=[-1 1 -1]
  Scope{,3,7,11..12,17..18} (7 alike) : Scope  NumInputPorts=4
  Scope1 : Scope  Commented=on  NumInputPorts=3
  Scope10 : Scope  Commented=on  NumInputPorts=2
  Scope2 : Scope  Commented=on  NumInputPorts=2
  Scope4 : Scope  Commented=on  NumInputPorts=3
  Scope5 : Scope  Commented=on  NumInputPorts=4
  Scope6 : Scope  NumInputPorts=2
  Scope8 : Scope  Commented=on  NumInputPorts=4
  Scope9 : Scope  NumInputPorts=2
  Sin : Trigonometry
  Sin1 : Trigonometry  Operator=cos
  Sin2 : Trigonometry  Commented=on
  Sum : Sum  Inputs=|-+
  Sum1 : Sum  Inputs=|-+
  Sum2 : Sum  Inputs=|+-
  Sum3 : Sum  Commented=on  Inputs=|-+
  Sum5 : Sum  Inputs=|-+
  Tan : Trigonometry  Commented=on  Operator=atan
  Terminator{,1..4} (5 alike) : Terminator
  Terminator5 : Terminator  Commented=on
  d_q : spsAlphaBetaZerotodq0Lib/Alpha-Beta-Zero to dq0  Alignment=Aligned with phase A axis
  d_q1 : spsAlphaBetaZerotodq0Lib/Alpha-Beta-Zero to dq0  Alignment=Aligned with phase A axis
  d_q2 : spsAlphaBetaZerotodq0Lib/Alpha-Beta-Zero to dq0  Commented=on  Alignment=Aligned with phase A axis
  dq0 to Alpha-Beta-Zero : spsdq0toAlphaBetaZeroLib/dq0 to Alpha-Beta-Zero  Alignment=Aligned with phase A axis
  Out1 : Outport
  Out2 : Outport  Port=2
  Out3 : Outport  Port=3
  Out4 : Outport  Port=4
  tag scope: S1=global, S2=global, S3=global, S4=global, Vref=global, ialpha=global, ibeta=global
  wires:
  Gain/1 -> [ialpha]
  d_q/1 -> Demux4/1
  Mux4/1 -> d_q/1
  First-Order Filter/1 -> First-Order Filter1/1
  First-Order Filter1/1 -> Gain/1
  Constant5/1 -> Mux4/3
  Demux2/3 -> Terminator1/1
  Demux4/3 -> Terminator/1
  Demux4/2 -> Sum/1, Scope17/4
  Constant1/1 -> Sum/2
  Demux4/1 -> Scope17/3, Sum1/1
  dq0 to Alpha-Beta-Zero/1 -> Demux1/1
  Demux1/3 -> Terminator2/1
  Demux1/2 -> [Vref], Scope9/2, Terminator3/1
  First-Order Filter2/1 -> First-Order Filter3/1
  First-Order Filter3/1 -> Gain2/1
  Mux2/1 -> d_q1/1
  Constant9/1 -> Mux2/3
  d_q1/1 -> Demux2/1
  Demux2/1 -> Scope18/3, Terminator4/1
  Demux2/2 -> Scope18/4, Sum5/1
  Constant10/1 -> Sum5/2
  Sum5/1 -> PID Controller3/1
  [wt] -> d_q/2
  [wt] -> dq0 to Alpha-Beta-Zero/2
  Sin1/1 -> Mux3/2, Scope/2
  Sin/1 -> Mux3/1
  Mux3/1 -> Scope/1
  PID Controller3/1 -> Scope/3, Scope/4, Sin1/1, Sin/1, [wt]
  Sum1/1 -> PID Controller4/1, Scope3/1
  Mux1/1 -> dq0 to Alpha-Beta-Zero/1
  Constant2/1 -> Mux1/3
  From15/1 -> Scope7/2
  From17/1 -> Scope7/4
  Logical Operator1/1 -> Goto2/1
  From32/1 -> GreaterThan1/1, GreaterThan/1, Scope10/1, Scope8/1, Mux/1
  GreaterThan1/1 -> Logical Operator1/1, Goto4/1
  Logical Operator/1 -> Goto1/1
  Pulse Generator1/1 -> Product1/2, Scope2/2
  Add1/1 -> Goto/1, Scope1/3
  From/1 -> GreaterThan/2, Scope10/2, Scope8/2, Mux/2
  GreaterThan/1 -> Goto3/1, Logical Operator/1
  Repeating Sequence/1 -> Product1/1, Product/2
  Product/1 -> Scope1/1, Add1/1
  Product1/1 -> Scope1/2, Add1/2
  From16/1 -> Scope7/3
  From14/1 -> Scope7/1
  Pulse Generator/1 -> Scope2/1, Product/1
  [ibeta] -> Scope17/2, Mux4/2
  [ialpha] -> Scope17/1, Mux4/1
  Mux/1 -> Scope8/4
  [ig] -> [ibeta], First-Order Filter/1
  Demux1/1 -> Scope9/1
  [wt] -> d_q1/2
  [Vg] -> Scope18/2, Mux2/2, First-Order Filter2/1
  Gain2/1 -> Scope18/1, Mux2/1
  PID Controller4/1 -> Mux1/1, Scope3/3
  PID Controller2/1 -> Mux1/2, Scope3/4
  Sum/1 -> Scope3/2, PID Controller2/1
  Divide/1 -> Tan/1
  Constant3/1 -> Divide2/2, Divide1/2
  Constant8/1 -> Divide2/1, Divide/2
  Product2/1 -> Scope4/3, Goto12/1
  Sin2/1 -> Scope4/1, Product2/1
  MATLAB Function/1(y) -> Scope4/2, Product2/2
  Sum3/1 -> Sin2/1
  Divide2/1 -> MATLAB Function/1(alpha)
  From5/1 -> Sum3/2
  Divide1/1 -> MATLAB Function/2(beta)
  Constant7/1 -> Divide/1, Divide1/1
  Tan/1 -> Sum3/1
  [Idref] -> Sum1/2
  Constant4/1 -> Mux5/3
  From1/1 -> d_q2/2
  Gain1/1 -> Scope5/1, Mux5/1
  Demux3/3 -> Terminator5/1
  First-Order Filter4/1 -> First-Order Filter5/1
  Mux5/1 -> d_q2/1
  From2/1 -> Mux5/2, Scope5/2, First-Order Filter4/1
  Demux3/1 -> Scope5/3, Goto7/1
  d_q2/1 -> Demux3/1
  Demux3/2 -> Goto5/1, Scope5/4
  First-Order Filter5/1 -> Gain1/1
  [Vdc] -> Sum2/1
  Constant6/1 -> Sum2/2
  Sum2/1 -> Scope6/1, PID Controller/1
  PID Controller/1 -> [Idref], Scope6/2
  Repeating Sequence1/1 -> Scope8/3, GreaterThan1/2
  Gain3/1 -> GreaterThan3/1, Mux6/3
  GreaterThan3/1 -> [S4], Out4/1, Scope12/3, Logical Operator3/1
  Logical Operator3/1 -> [S3], Out3/1, Scope12/4
  Logical Operator2/1 -> Out2/1, Scope12/2, [S2]
  Mux6/1 -> Scope11/4
  Repeating Sequence2/1 -> GreaterThan3/2, Scope11/3, Mux6/2, Scope11/2, GreaterThan2/2
  GreaterThan2/1 -> Logical Operator2/1, Out1/1, Scope12/1, [S1]
  [Vref] -> GreaterThan2/1, Gain3/1, Mux6/1, Scope11/1

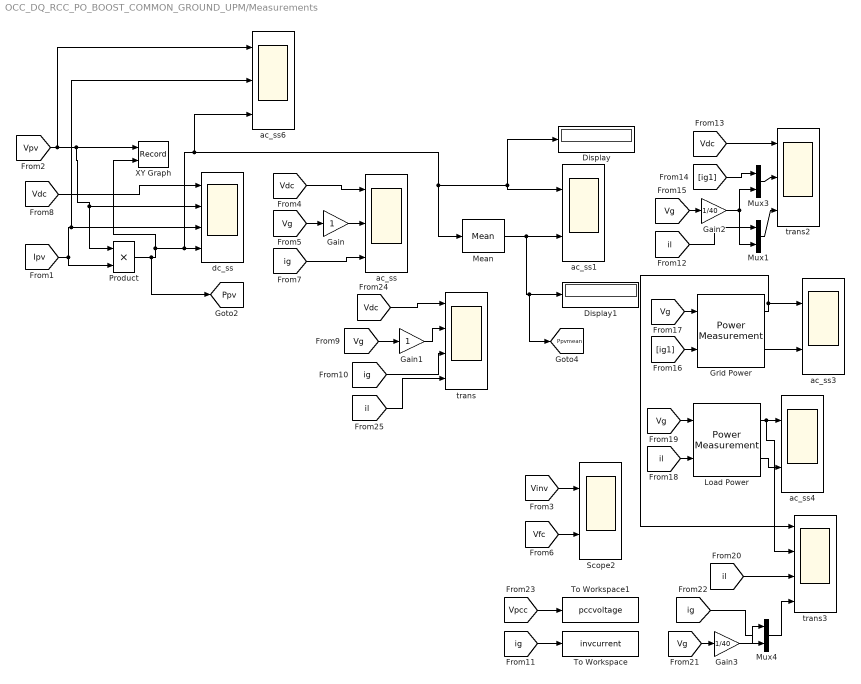
== system OCC_DQ_RCC_PO_BOOST_COMMON_GROUND_UPM/Measurements ==
  Display : Display
  Display1 : Display
  Gain : Gain
  Gain1 : Gain
  Gain2 : Gain  Gain=1/40
  Gain3 : Gain  Gain=1/40
  Grid Power : eePowerMeasurement/Power Measurement  LabelModeActiveChoice=Continuous  F=50  K=[1]  Ts=0
  Load Power : eePowerMeasurement/Power Measurement  LabelModeActiveChoice=Continuous  F=50  K=[1]  Ts=0
  Mean : spsMeanLib/Mean  Freq=50  Vinit=0  Ts=1e-6
  Mux1 : Mux  Inputs=2
  Mux3 : Mux  Inputs=2
  Mux4 : Mux  Inputs=2
  Product : Product
  Scope2 : Scope  NumInputPorts=2
  To Workspace : ToWorkspace  VariableName=invcurrent  SaveFormat=Structure With Time  SampleTime=-1
  To Workspace1 : ToWorkspace  VariableName=pccvoltage  SaveFormat=Structure With Time  SampleTime=-1
  XY Graph : Record  FileSettingsInternal="{\"entries\":[{\"content\":{\"excelSettings\":{\"content\":{},\"type\":\"Streamout.ExcelSettings\"}},\"type\":\"Streamout.FileSettingStorage\",\"uuid\":\"\"}],\"packageUris\":[\"http:\\/\\/schema.mathworks.com\\/mf0\\/streamout_blocks\\/R2020a\"],\"version\":\"1.0\"}"  Layout=[1 1]  SignalsInternal="{\"entries\":[{\"content\":{\"signals\":[{\"content\":{\"blockPath\":[],\"dimensions\":[1],\"domain\":\"\",\"lineColor\":\"#b746ff\",\"port\":1,\"sid\":[\"\"],\"signalID\":2575,\"signalName\":\"From2\"},\"type\":\"RecordBlkView.Signal\",\"uuid\":\"\"},{\"content\":{\"blockPath\":[],\"dimensions\":[1],\"domain\":\"\",\"lineColor\":\"#d95319\",\"plots\":[1],\"port\":2,\"sid\":[\"\"],\"signalID\":2579,\"signalName\":\"Product\"},\"type\":\"RecordBlkView.Signal\",\"uuid\":\"\"}]},\"type\":\"RecordBlkView.InputSignals\",\"uuid\":\"\"}],\"packageUris\":[\"http:\\/\\/schema.mathworks.com\\/mf0\\/streamout_blocks\\/R2020a\"],\"version\":\"1.0\"}"  VisualizationBindings="{\"xyplotplugin\":{\"info\":[{\"series\":[{\"bindingParametersList\":[{\"parameter\":\"Y-Axis\",\"signalID\":2579,\"signalName\":\"Product\"}],\"seriesID\":41862}],\"subplotID\":1}]}}"  CompatibilityTag=XY
  ac_ss : Scope  NumInputPorts=3
  ac_ss1 : Scope  NumInputPorts=2
  ac_ss3 : Scope  NumInputPorts=2
  ac_ss4 : Scope  NumInputPorts=2
  ac_ss6 : Scope  NumInputPorts=3
  dc_ss : Scope  NumInputPorts=4
  trans : Scope  NumInputPorts=4
  trans2 : Scope  NumInputPorts=3
  trans3 : Scope  NumInputPorts=4
  tag scope: Ppv=global, Ppvmean=global
  wires:
  Mean/1 -> ac_ss1/2, [Ppvmean], Display1/1
  Gain2/1 -> Mux3/2, Mux1/2
  Gain/1 -> ac_ss/2
  Product/1 -> [Ppv], ac_ss6/3, Display/1, ac_ss1/1, Mean/1, dc_ss/4, XY Graph/2
  [ig] -> To Workspace/1
  [Vdc] -> ac_ss/1
  Grid Power/2 -> ac_ss3/2
  [il] -> trans/4
  [Vdc] -> dc_ss/1
  [il] -> Mux1/1
  [il] -> Load Power/2
  [ig] -> Mux4/2
  [Vg] -> Gain3/1
  [Vdc] -> trans/1
  Mux1/1 -> trans2/3
  [ig] -> ac_ss/3
  [Vg] -> Gain/1
  [Vg] -> Gain1/1
  Gain1/1 -> trans/2
  [Vpv] -> ac_ss6/1, dc_ss/2, Product/1, XY Graph/1
  [Vg] -> Load Power/1
  [Vpcc] -> To Workspace1/1
  Mux4/1 -> trans3/4
  [Vdc] -> trans2/1
  [Vg] -> Gain2/1
  [Vfc] -> Scope2/2
  Grid Power/1 -> trans3/1, ac_ss3/1
  [ig1] -> Grid Power/2
  Load Power/1 -> trans3/2, ac_ss4/1
  Load Power/2 -> ac_ss4/2
  [ig1] -> Mux3/1
  [Ipv] -> ac_ss6/2, dc_ss/3, Product/2
  [ig] -> trans/3
  Mux3/1 -> trans2/2
  Gain3/1 -> Mux4/1
  [Vg] -> Grid Power/1
  [il] -> trans3/3
  [Vinv] -> Scope2/1

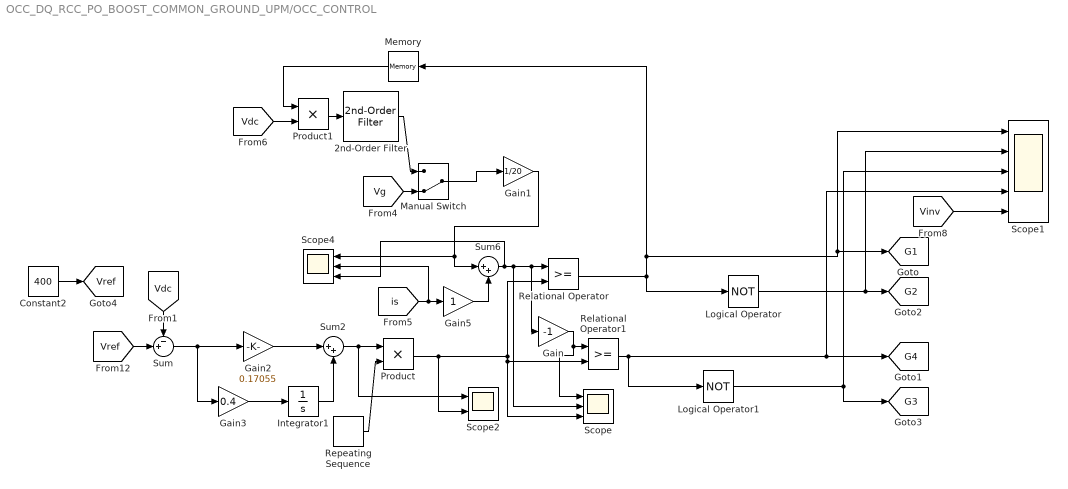
== system OCC_DQ_RCC_PO_BOOST_COMMON_GROUND_UPM/OCC_CONTROL ==
  2nd-Order Filter : powerlib_extras/Control  Blocks/2nd-Order Filter  FilterType=Bandpass  Fo=50  Zeta=0.25  Initialize=off  Vac_Init=[1 45 60]  Vdc_Init=-0.5  PlotResponse=off  param1=[1 500 1]
  Constant2 : Constant  Value=400
  Gain : Gain  Gain=-1
  Gain1 : Gain  Gain=1/20
  Gain2 : Gain  Gain=0.17055
  Gain3 : Gain  Gain=0.4
  Gain5 : Gain
  Integrator1 : Integrator  UpperSaturationLimit=120  LowerSaturationLimit=0
  Logical Operator : Logic  Operator=NOT  AllPortsSameDT=off  OutDataTypeStr=boolean
  Logical Operator1 : Logic  Operator=NOT  AllPortsSameDT=off  OutDataTypeStr=boolean
  Manual Switch : ManualSwitch  CurrentSetting=0
  Memory : Memory
  Product : Product
  Product1 : Product  RndMeth=Zero
  Relational Operator : RelationalOperator  OutDataTypeStr=boolean  RndMeth=Simplest  InputSameDT=off
  Relational Operator1 : RelationalOperator  OutDataTypeStr=boolean  RndMeth=Simplest  InputSameDT=off
  Repeating Sequence : simulink/Sources/Repeating Sequence  rep_seq_t=[0 0.5 1]*(1/10000)  rep_seq_y=[-1 1 -1]
  Scope : Scope  NumInputPorts=3
  Scope1 : Scope  NumInputPorts=5
  Scope2 : Scope  NumInputPorts=2
  Scope4 : Scope  NumInputPorts=3
  Sum : Sum  Inputs=-+|
  Sum2 : Sum  Inputs=|++
  Sum6 : Sum  Inputs=|++
  tag scope: G1=global, G2=global, G3=global, G4=global, Vref=global
  wires:
  Sum/1 -> Gain3/1, Gain2/1
  Memory/1 -> Product1/1
  Gain5/1 -> Sum6/2
  Product1/1 -> 2nd-Order Filter/1
  Product/1 -> Scope2/2, Scope/3, Relational Operator1/2, Relational Operator/2
  Sum6/1 -> Scope4/3, Scope/2, Gain/1, Relational Operator/1
  [Vdc] -> Sum/1
  [is] -> Scope4/2, Gain5/1
  Gain1/1 -> Scope4/1, Sum6/1
  [Vref] -> Sum/2
  Gain3/1 -> Integrator1/1
  Sum2/1 -> Scope2/1, Product/1
  Constant2/1 -> [Vref]
  Gain2/1 -> Sum2/1
  Repeating Sequence/1 -> Product/2
  Integrator1/1 -> Sum2/2
  [Vdc] -> Product1/2
  Gain/1 -> Scope/1, Relational Operator1/1
  Logical Operator1/1 -> Scope1/3, [G3]
  Relational Operator/1 -> Logical Operator/1, Scope1/1, [G1], Memory/1
  Logical Operator/1 -> Scope1/2, [G2]
  [Vinv] -> Scope1/5
  Manual Switch/1 -> Gain1/1
  2nd-Order Filter/1 -> Manual Switch/1
  [Vg] -> Manual Switch/2
  Relational Operator1/1 -> Logical Operator1/1, [G4], Scope1/4
